simulink model "afe_dq_ttype"  (R2026b)
settings: Solver=ode23tb  StopTime=param.sim.simlength  FixedStep=param.sim.tc  MaxStep=param.glb_time.tc
values from neighbouring files (symbols this model uses):
  param = struct()    [init_model.m]
undefined symbols (not defined in the file or in its folder): magnitude
libraries: fl_lib x281, nesl_utility x136, igbt_simple_2th_lib x12, single_phase_transformer_lib x3, discrete_time_low_pass_filter x1, threephase_inductor_lib x1, dclink_for_three_levels x1, three_phase_three_level_ttype_inverter_ideal_switch_based_model x1, three_phase_three_levels_PWM_modulator x1, three_phase_bridge_three_level_ttype_igbt_simple_2th x1, three_phase_voltage_with_frt_emulator_mfcn x1
(part 8 of 8)

== system afe_dq_ttype/afe_dq_mod1/AFE_control/afe_control/grid_voltage_phase_lock_loops/FHT-PLL/pll_stageA/filter_and_transformation/FHTbeta ==
  u : Inport
  Bus Selector : BusSelector  OutputSignals=output_pu_hat,output_pu_hat_dot
  C Caller : CCaller  FunctionName=first_harmonic_tracker_process_simulink  PortSpecificationStruct="%)30     .    B \\   8    (     @         %    \"     D    !     0         %  0 \"0    $    _    07)G3F%M90  4&]R=$YA;64 4V-O<&4     26YD97@     5'EP90      4VEZ90      27-';&]B86P   X    P    !@    @    $          4    (     0    ,    !         !   P!O=70 #@   #     &    \"     0         !0    @    !     P    $         $  # &]U=  .    .     8    (    !          %    \"     $    &     0         0  ...(+4988 chars)"
  Constant : Constant  Value=param.glb_time.ts_afe
  Constant1 : Constant  Value=14
  Constant4 : Constant  Value=param.afe.ctrl.fht.omega_fht
  Constant5 : Constant  Value=param.afe.ctrl.fht.delta_fht
  Constant6 : Constant  Value=param.afe.ctrl.fht.Ld_fht(1)
  Constant7 : Constant  Value=param.afe.ctrl.fht.Ld_fht(2)
  Data Type Conversion{1..2,6..9} (6 alike) : DataTypeConversion  OutDataTypeStr=single  SaturateOnIntegerOverflow=off  RndMeth=Floor
  Data Type Conversion10 : DataTypeConversion  OutDataTypeStr=double  SaturateOnIntegerOverflow=off  RndMeth=Floor
  Data Type Conversion3 : DataTypeConversion  OutDataTypeStr=uint8  SaturateOnIntegerOverflow=off  RndMeth=Floor
  Data Type Conversion4 : DataTypeConversion  OutDataTypeStr=double  SaturateOnIntegerOverflow=off  RndMeth=Floor
  Data Type Conversion5 : DataTypeConversion  OutDataTypeStr=uint8  SaturateOnIntegerOverflow=off  RndMeth=Floor
  Gain : Gain  Gain=1/param.afe.ctrl.fht.omega_fht
  Step : Step  Time=0.0125  InitialValue=1  FinalValue=0
  ud_hat : Outport
  uq_hat : Outport  Port=2
  wires:
  Gain/1 -> uq_hat/1
  Bus Selector/2 -> Data Type Conversion10/1  "<output_pu_hat_dot>"
  Data Type Conversion10/1 -> Gain/1
  Data Type Conversion4/1 -> ud_hat/1
  Data Type Conversion3/1 -> C Caller/1
  Data Type Conversion1/1 -> C Caller/3
  Data Type Conversion2/1 -> C Caller/2
  C Caller/1 -> Bus Selector/1
  Bus Selector/1 -> Data Type Conversion4/1  "<output_pu_hat>"
  Step/1 -> Data Type Conversion3/1
  u/1 -> Data Type Conversion2/1
  Constant/1 -> Data Type Conversion1/1
  Constant1/1 -> Data Type Conversion5/1
  Constant4/1 -> Data Type Conversion6/1
  Constant6/1 -> Data Type Conversion8/1
  Constant7/1 -> Data Type Conversion9/1
  Constant5/1 -> Data Type Conversion7/1
  Data Type Conversion5/1 -> C Caller/8
  Data Type Conversion6/1 -> C Caller/4
  Data Type Conversion7/1 -> C Caller/5
  Data Type Conversion8/1 -> C Caller/6
  Data Type Conversion9/1 -> C Caller/7

== system afe_dq_ttype/afe_dq_mod1/AFE_control/afe_control/grid_voltage_phase_lock_loops/FHT-PLL_simulink/pll_stageA/filter_and_transformation/FHTalpha ==
  u : Inport
  Gain : Gain  Gain=param.afe.ctrl.fht.Ld_fht  Multiplication=Matrix(K*u)
  Gain1 : Gain  Gain=param.afe.ctrl.fht.Ad_fht  Multiplication=Matrix(K*u)
  Gain2 : Gain  Gain=param.afe.ctrl.fht.Cfht  Multiplication=Matrix(K*u)
  Gain3 : Gain  Gain=1/param.afe.ctrl.fht.omega_fht
  Selector : Selector  InputPortWidth=2  IndexOptions=Index vector (dialog)  Indices=1  OutputSizes=1  RuntimeRangeChecks=off
  Selector1 : Selector  InputPortWidth=2  IndexOptions=Index vector (dialog)  Indices=2  OutputSizes=1  RuntimeRangeChecks=off
  Sum : Sum  Inputs=-+|
  Sum1 : Sum  Inputs=|++
  Unit Delay : UnitDelay  SampleTime=-1
  ualpha : Outport
  ubeta : Outport  Port=2
  wires:
  u/1 -> Sum/2
  Unit Delay/1 -> Gain2/1, Selector1/1, Selector/1, Gain1/1
  Sum/1 -> Gain/1
  Sum1/1 -> Unit Delay/1
  Gain1/1 -> Sum1/2
  Gain2/1 -> Sum/1
  Selector/1 -> ualpha/1
  Gain/1 -> Sum1/1
  Selector1/1 -> Gain3/1
  Gain3/1 -> ubeta/1

== system afe_dq_ttype/afe_dq_mod1/AFE_control/afe_control/grid_voltage_phase_lock_loops/FHT-PLL_simulink/pll_stageA/filter_and_transformation/FHTbeta ==
  u : Inport
  Gain : Gain  Gain=param.afe.ctrl.fht.Ld_fht  Multiplication=Matrix(K*u)
  Gain1 : Gain  Gain=param.afe.ctrl.fht.Ad_fht  Multiplication=Matrix(K*u)
  Gain2 : Gain  Gain=param.afe.ctrl.fht.Cfht  Multiplication=Matrix(K*u)
  Gain3 : Gain  Gain=1/param.afe.ctrl.fht.omega_fht
  Selector : Selector  InputPortWidth=2  IndexOptions=Index vector (dialog)  Indices=1  OutputSizes=1  RuntimeRangeChecks=off
  Selector1 : Selector  InputPortWidth=2  IndexOptions=Index vector (dialog)  Indices=2  OutputSizes=1  RuntimeRangeChecks=off
  Sum : Sum  Inputs=-+|
  Sum1 : Sum  Inputs=|++
  Unit Delay : UnitDelay  SampleTime=-1
  ualpha : Outport
  ubeta : Outport  Port=2
  wires:
  Gain3/1 -> ubeta/1
  Selector1/1 -> Gain3/1
  Gain/1 -> Sum1/1
  Selector/1 -> ualpha/1
  Gain2/1 -> Sum/1
  Gain1/1 -> Sum1/2
  Sum1/1 -> Unit Delay/1
  Sum/1 -> Gain/1
  Unit Delay/1 -> Gain1/1, Selector/1, Selector1/1, Gain2/1
  u/1 -> Sum/2

== system afe_dq_ttype/afe_dq_mod1/AFE_control/afe_control/grid_voltage_phase_lock_loops/dq_pll/pll_stageA/sequences/alphabeta2xieta ==
  alpha : Inport
  beta : Inport  Port=2
  gamma : Inport  Port=3
  alphabeta2xieta_neg : MATLAB Function  TreatAsAtomicUnit=on
  alphabeta2xieta_pos : MATLAB Function  TreatAsAtomicUnit=on
  xi : Outport
  eta : Outport  Port=2
  Out3 : Outport  Port=3
  Out4 : Outport  Port=4
  wires:
  alpha/1 -> alphabeta2xieta_neg/1(alpha), alphabeta2xieta_pos/1(alpha)  "u_grid_alpha"
  beta/1 -> alphabeta2xieta_neg/2(beta), alphabeta2xieta_pos/2(beta)  "u_grid_beta"
  gamma/1 -> alphabeta2xieta_neg/3(gamma), alphabeta2xieta_pos/3(gamma)  "phase_grid"
  alphabeta2xieta_pos/1(xi) -> xi/1  "u_grid_pos_xi"
  alphabeta2xieta_pos/2(eta) -> eta/1  "u_grid_pos_eta"
  alphabeta2xieta_neg/1(xi) -> Out3/1  "u_grid_neg_xi"
  alphabeta2xieta_neg/2(eta) -> Out4/1  "u_grid_neg_eta"

== matlab function afe_dq_ttype/afe_dq_mod1/AFE_control/afe_control/grid_voltage_phase_lock_loops/FHT-PLL_simulink/pll_stageA/filter_and_transformation/abc2alphabeta ==
  data: a input; alpha output; b input; c input; beta output
function [alpha,beta] = abc2alphabeta(a,b,c)

alpha = 2/3*(a - 1/2*b - 1/2*c);
beta  = 1/sqrt(3)*(b - c);

end

== matlab function afe_dq_ttype/afe_dq_mod1/AFE_control/afe_control/grid_voltage_phase_lock_loops/FHT-PLL_simulink/pll_stageA/sequences/alphabeta2xieta ==
  data: alpha input; xi output; beta input; gamma input; eta output
function [xi,eta] = alphabeta2xieta_pos(alpha,beta,gamma)

    xi  =  (alpha*cos(gamma) + beta*sin(gamma));
    eta = (-alpha*sin(gamma) + beta*cos(gamma));

end

== matlab function afe_dq_ttype/afe_dq_mod1/AFE_control/afe_control/grid_voltage_phase_lock_loops/FHT-PLL_simulink/pll_stageB/bounder1 ==
  data: u input; y output
function y = bounder(u)
    y = -pi + mod(u+3*pi,2*pi);
end

== matlab function afe_dq_ttype/afe_dq_mod1/AFE_control/afe_control/grid_voltage_phase_lock_loops/FHT-PLL_simulink/pll_stageB/double_integrator_observer/bounder1 ==
  data: u input; y output
function y = bounder(u)
    
    y = -pi + mod(u+3*pi,2*pi);
    
end

== matlab function afe_dq_ttype/afe_dq_mod1/AFE_control/afe_control/grid_voltage_phase_lock_loops/dq_pll/pll_stageA/mormalization_and_transformation/abc2alphabeta ==
  data: a input; alpha output; b input; c input; beta output
function [alpha,beta] = abc2alphabeta(a,b,c)

alpha = 2/3*(a - 1/2*b - 1/2*c);
beta  = 1/sqrt(3)*(b - c);

end

== matlab function afe_dq_ttype/afe_dq_mod1/AFE_control/afe_control/grid_voltage_phase_lock_loops/dq_pll/pll_stageA/sequences/alphabeta2xieta/alphabeta2xieta_neg ==
  data: alpha input; xi output; beta input; gamma input; eta output
function [xi,eta] = alphabeta2xieta_neg(alpha,beta,gamma)

    xi  = alpha*cos(gamma) - beta*sin(gamma);
    eta = alpha*sin(gamma) + beta*cos(gamma);

end

== matlab function afe_dq_ttype/afe_dq_mod1/AFE_control/afe_control/grid_voltage_phase_lock_loops/dq_pll/pll_stageA/sequences/alphabeta2xieta/alphabeta2xieta_pos ==
  data: alpha input; xi output; beta input; gamma input; eta output
function [xi,eta] = alphabeta2xieta_pos(alpha,beta,gamma)

    xi  =  alpha*cos(gamma) + beta*sin(gamma);
    eta = -alpha*sin(gamma) + beta*cos(gamma);

end

== matlab function afe_dq_ttype/afe_dq_mod1/AFE_control/afe_control/grid_voltage_phase_lock_loops/dq_pll/pll_stageB/double_integrator_observer/bounder1 ==
  data: u input; y output
function y = bounder(u)
    
    y = -pi + mod(u+3*pi,2*pi);
    
end

== matlab function afe_dq_ttype/afe_dq_mod1/AFE_control/afe_control/grid_voltage_phase_lock_loops/dq_pll/pll_stageB/double_integrator_observer/bounder2 ==
  data: u input; y output
function y = bounder(u)
    
    y = -pi + mod(u+3*pi,2*pi);
    
end

== matlab function afe_dq_ttype/grid/power meter iec mfunc/three_phase_power_meter_iec ==
  data: phase input; m output Bus: PowerMeterIecBus; u_abc input; i_abc input; omega input; ts input; enable_time input
function m = three_phase_power_meter_iec(phase, u_abc, i_abc, omega, ts, enable_time)
%#codegen
% THREE_PHASE_POWER_METER_IEC
% Equivalente in singolo blocco MATLAB Function del sottosistema Simulink
% "three_phase_power_meter_iec" (libreria power_meter_iec).
%
% INGRESSI
%   phase       : angolo del PLL [rad]      (scalare)
%   u_abc       : tensioni di fase [V]      (3x1)
%   i_abc       : correnti di linea [A]     (3x1)
%   omega       : pulsazione di rete [rad/s] (scalare)
%   ts          : passo di campionamento [s]  -> parametro di maschera
%   enable_time : istante di abilitazione [s] -> parametro di maschera
%
% USCITA
%   m : struct (bus) con i campi, nello stesso ordine del Bus Creator
%       originale: Q1p, Q1n, P1n, P1p, U1n, U1p,
%                  i_act_1n, i_react_1n, i_act_1p, i_react_1p
%
% CATENA DI ELABORAZIONE (identica all'originale)
%   1) proiezione di ogni fase su cos(phase) e sin(phase), guadagno 2
%   2) media mobile dinamica su finestra pari a mezzo periodo di rete
%      (Tw = pi/|omega|), con lunghezza frazionaria interpolata
%   3) componenti simmetriche di sequenza diretta e inversa (Fortescue)
%   4) potenze attiva e reattiva per sequenza, tensioni concatenate RMS,
%      correnti attiva e reattiva per sequenza
%
% NOTE
%   - Il blocco deve girare a passo fisso ts (gli Zero-Order Hold di
%     ingresso dell'originale sono impliciti nel sample time del blocco).
%   - ts ed enable_time possono essere dichiarati come dati di scope
%     "Parameter" nel Symbols pane del MATLAB Function block, cosi'
%     risolvono direttamente sui parametri di maschera e la firma
%     esterna resta a 4 ingressi come nel blocco originale.

% ------------------------------------------------------------------
% Costanti
% ------------------------------------------------------------------
% MAVGFLT_SIZE_MAX = 17500;   % lunghezza buffer circolare (come originale)
MAVGFLT_SIZE_MAX = 2048;   % lunghezza buffer ridotto
NCH              = 12;      % canali filtrati: 6 per u_abc, 6 per i_abc

% Ordine canali:
%   1..3  ua_cos ub_cos uc_cos      7..9   ia_cos ib_cos ic_cos
%   4..6  ua_sin ub_sin uc_sin     10..12  ia_sin ib_sin ic_sin

% ------------------------------------------------------------------
% Stato persistente
% ------------------------------------------------------------------
persistent buf cb_index sample_count sum_short sum_long prev_input ...
           k_step period_held

if isempty(buf)
    buf          = zeros(NCH, MAVGFLT_SIZE_MAX);
    cb_index     = ones(NCH, 1);
    sample_count = ones(NCH, 1);
    sum_short    = zeros(NCH, 1);
    sum_long     = zeros(NCH, 1);
    prev_input   = zeros(NCH, 1);
    k_step       = 0;
    period_held  = 0;          % uscita iniziale dell'Enabled Subsystem
end

% ------------------------------------------------------------------
% Abilitazione (equivalente al blocco Step con Time = enable_time)
% ------------------------------------------------------------------
t_now  = k_step * ts;
k_step = k_step + 1;
enable = (t_now >= enable_time);

% ------------------------------------------------------------------
% Finestra di media: Enabled Subsystem 2*pi/w, alimentato da 2*|omega|.
% Quando |omega| = 0 l'Enabled Subsystem mantiene l'ultimo valore.
% ------------------------------------------------------------------
w2 = 2 * abs(omega);
if w2 > 0
    period_held = 2*pi / w2;   % = pi/|omega|, mezzo periodo di rete
end
period = period_held;

% ------------------------------------------------------------------
% Proiezione sin/cos, guadagno 2
% ------------------------------------------------------------------
c = cos(phase);
s = sin(phase);

x = zeros(NCH, 1);
x(1)  = 2 * u_abc(1) * c;   x(2)  = 2 * u_abc(2) * c;   x(3)  = 2 * u_abc(3) * c;
x(4)  = 2 * u_abc(1) * s;   x(5)  = 2 * u_abc(2) * s;   x(6)  = 2 * u_abc(3) * s;
x(7)  = 2 * i_abc(1) * c;   x(8)  = 2 * i_abc(2) * c;   x(9)  = 2 * i_abc(3) * c;
x(10) = 2 * i_abc(1) * s;   x(11) = 2 * i_abc(2) * s;   x(12) = 2 * i_abc(3) * s;

% ------------------------------------------------------------------
% Banco di 12 filtri a media mobile dinamica (dmavgflt_process)
% ------------------------------------------------------------------
y = zeros(NCH, 1);

if enable && period > 0

    desired = period / ts;
    if desired > (MAVGFLT_SIZE_MAX - 1)
        desired = MAVGFLT_SIZE_MAX - 1;
    end

    n_samples = floor(desired + 1);          % campioni che coprono il periodo
    frac      = desired + 1 - n_samples;     % parte frazionaria
    if n_samples < 1
        n_samples = 1;
    end

    for ch = 1:NCH

        ci = cb_index(ch);
        sc = sample_count(ch);

        if n_samples > sc
            % finestra in crescita: aggiungi campioni
            sum_short(ch) = sum_short(ch) + prev_input(ch);
            sum_long(ch)  = sum_long(ch)  + x(ch);
            sc = sc + 1;

        elseif n_samples < sc
            % finestra in contrazione: rimuovi i due campioni piu' vecchi
            i1 = mod(ci - 1 - sc,       MAVGFLT_SIZE_MAX) + 1;
            i2 = mod(ci - 1 - (sc - 1), MAVGFLT_SIZE_MAX) + 1;
            old_sum = buf(ch, i1) + buf(ch, i2);

            sum_short(ch) = sum_short(ch) + prev_input(ch) - old_sum;
            sum_long(ch)  = sum_long(ch)  + x(ch)          - old_sum;
            sc = sc - 1;

        else
            % finestra costante
            i1     = mod(ci - 1 - sc, MAVGFLT_SIZE_MAX) + 1;
            oldest = buf(ch, i1);

            sum_short(ch) = sum_short(ch) + prev_input(ch) - oldest;
            sum_long(ch)  = sum_long(ch)  + x(ch)          - oldest;
        end

        % aggiornamento buffer circolare
        buf(ch, ci)      = x(ch);
        cb_index(ch)     = mod(ci, MAVGFLT_SIZE_MAX) + 1;
        prev_input(ch)   = x(ch);
        sample_count(ch) = sc;

        % uscita: interpolazione lineare fra finestra corta e lunga
        if sc > 1
            avg_short = sum_short(ch) / (sc - 1);
        else
            avg_short = 0;
        end
        avg_long = sum_long(ch) / sc;

        y(ch) = avg_short * (1 - frac) + avg_long * frac;
    end
end
% se enable = false oppure period <= 0: y resta 0 e lo stato non evolve
% (comportamento identico all'originale)

ua_cos = y(1);  ub_cos = y(2);  uc_cos = y(3);
ua_sin = y(4);  ub_sin = y(5);  uc_sin = y(6);
ia_cos = y(7);  ib_cos = y(8);  ic_cos = y(9);
ia_sin = y(10); ib_sin = y(11); ic_sin = y(12);

% ------------------------------------------------------------------
% Componenti simmetriche (fasori con convenzione U = u_cos - j*u_sin)
% ------------------------------------------------------------------
sq3 = sqrt(3);

u1p_cos = (2*ua_cos - ub_cos - uc_cos - sq3*(uc_sin - ub_sin)) / 6;
u1p_sin = (2*ua_sin - ub_sin - uc_sin - sq3*(ub_cos - uc_cos)) / 6;
u1n_cos = (2*ua_cos - ub_cos - uc_cos - sq3*(ub_sin - uc_sin)) / 6;
u1n_sin = (2*ua_sin - ub_sin - uc_sin - sq3*(uc_cos - ub_cos)) / 6;

i1p_cos = (2*ia_cos - ib_cos - ic_cos - sq3*(ic_sin - ib_sin)) / 6;
i1p_sin = (2*ia_sin - ib_sin - ic_sin - sq3*(ib_cos - ic_cos)) / 6;
i1n_cos = (2*ia_cos - ib_cos - ic_cos - sq3*(ib_sin - ic_sin)) / 6;
i1n_sin = (2*ia_sin - ib_sin - ic_sin - sq3*(ic_cos - ib_cos)) / 6;

% ------------------------------------------------------------------
% Potenze per sequenza
% ------------------------------------------------------------------
P1p = 1.5 * (u1p_cos*i1p_cos + u1p_sin*i1p_sin);
Q1p = 1.5 * (u1p_cos*i1p_sin - u1p_sin*i1p_cos);
P1n = 1.5 * (u1n_cos*i1n_cos + u1n_sin*i1n_sin);
Q1n = 1.5 * (u1n_cos*i1n_sin - u1n_sin*i1n_cos);

% ------------------------------------------------------------------
% Tensioni concatenate RMS per sequenza: sqrt(3/2)*ampiezza di fase
% ------------------------------------------------------------------
U1p = sqrt(1.5 * (u1p_cos^2 + u1p_sin^2));
U1n = sqrt(1.5 * (u1n_cos^2 + u1n_sin^2));

% ------------------------------------------------------------------
% Correnti attiva e reattiva per sequenza (RMS di linea)
% La protezione contro la divisione per zero non era presente nello
% schema originale (i blocchi Divide restituivano Inf/NaN a U = 0).
% Portare U_MIN a 0 per replicare esattamente il comportamento vecchio.
% ------------------------------------------------------------------
U_MIN = 1e-9;

if U1p > U_MIN
    i_act_1p   = P1p / (sq3 * U1p);
    i_react_1p = Q1p / (sq3 * U1p);
else
    i_act_1p   = 0;
    i_react_1p = 0;
end

if U1n > U_MIN
    i_act_1n   = P1n / (sq3 * U1n);
    i_react_1n = Q1n / (sq3 * U1n);
else
    i_act_1n   = 0;
    i_react_1n = 0;
end

% ------------------------------------------------------------------
% Bus di uscita (stesso ordine dei campi dell'originale)
% ------------------------------------------------------------------
m.Q1p        = Q1p;
m.Q1n        = Q1n;
m.P1n        = P1n;
m.P1p        = P1p;
m.U1n        = U1n;
m.U1p        = U1p;
m.i_act_1n   = i_act_1n;
m.i_react_1n = i_react_1n;
m.i_act_1p   = i_act_1p;
m.i_react_1p = i_react_1p;

end

== matlab function afe_dq_ttype/afe_dq_mod1/AFE_control/afe_control/current_ctrl/xi_eta_to_alpha_beta ==
  data: xi input; alpha output; eta input; phase input; beta output
function [alpha,beta] = xi_eta_to_alpha_beta(xi,eta,phase)

    alpha = xi*cos(phase) - eta*sin(phase);
    beta  = xi*sin(phase) + eta*cos(phase);

end

== matlab function afe_dq_ttype/afe_dq_mod1/AFE_control/afe_control/grid_voltage_phase_lock_loops/dq_pll/pll_stageB/bounder1 ==
  data: u input; y output
function y = bounder(u)
    y = -pi + mod(u+3*pi,2*pi);
end

== matlab function afe_dq_ttype/afe_dq_mod1/AFE_control/afe_control/grid_voltage_phase_lock_loops/FHT-PLL_simulink/pll_stageB/double_integrator_observer/bounder2 ==
  data: u input; y output
function y = bounder(u)
    
    y = -pi + mod(u+3*pi,2*pi);
    
end

== matlab function afe_dq_ttype/afe_dq_mod1/afe/deadtime_generator_for_ttype/dead_time_generator_cmos_simulink_phu/dead_time_leg_generator_1/MATLAB Function ==
  data: u input; y output; Vpos_rail_dtg parameter
function y = not_cmos(u, Vpos_rail_dtg)

vth = Vpos_rail_dtg/2;

if u > vth
    y = 0;
else
    y = Vpos_rail_dtg;
end

== matlab function afe_dq_ttype/afe_dq_mod1/afe/deadtime_generator_for_ttype/dead_time_generator_cmos_simulink_phu/dead_time_leg_generator_1/MATLAB Function1 ==
  data: u1 input; u2 input; y output; Vpos_rail_dtg parameter
function y = and_cmos(u1, u2, Vpos_rail_dtg)

vth = Vpos_rail_dtg/2;

if (u1 > vth && u2 > vth)
    y = Vpos_rail_dtg;
else
    y = 0;
end

== matlab function afe_dq_ttype/afe_dq_mod1/afe/deadtime_generator_for_ttype/dead_time_generator_cmos_simulink_phu/dead_time_leg_generator_1/MATLAB Function2 ==
  data: u input; y output; Vpos_rail_dtg parameter
function y = not_cmos(u, Vpos_rail_dtg)

vth = Vpos_rail_dtg/2;

if u > vth
    y = 0;
else
    y = Vpos_rail_dtg;
end

== matlab function afe_dq_ttype/afe_dq_mod1/afe/deadtime_generator_for_ttype/dead_time_generator_cmos_simulink_phu/dead_time_leg_generator_1/MATLAB Function3 ==
  data: u input; y output; Vpos_rail_dtg parameter
function y = not_cmos(u, Vpos_rail_dtg)

vth = Vpos_rail_dtg/2;

if u > vth
    y = 0;
else
    y = Vpos_rail_dtg;
end

== matlab function afe_dq_ttype/afe_dq_mod1/afe/deadtime_generator_for_ttype/dead_time_generator_cmos_simulink_phu/dead_time_leg_generator_1/MATLAB Function4 ==
  data: u1 input; u2 input; y output; Vpos_rail_dtg parameter
function y = and_cmos(u1, u2, Vpos_rail_dtg)

vth = Vpos_rail_dtg/2;

if (u1 > vth && u2 > vth)
    y = Vpos_rail_dtg;
else
    y = 0;
end

== matlab function afe_dq_ttype/afe_dq_mod1/afe/deadtime_generator_for_ttype/dead_time_generator_cmos_simulink_phu/dead_time_leg_generator_1/MATLAB Function5 ==
  data: u1 input; u2 input; y output; Vpos_rail_dtg parameter
function y = and_cmos(u1, u2, Vpos_rail_dtg)

vth = Vpos_rail_dtg/2;

if (u1 > vth && u2 > vth)
    y = Vpos_rail_dtg;
else
    y = 0;
end

== matlab function afe_dq_ttype/afe_dq_mod1/afe/deadtime_generator_for_ttype/dead_time_generator_cmos_simulink_phu/dead_time_leg_generator_1/MATLAB Function6 ==
  data: u input; y output; Vpos_rail_dtg parameter
function y = not_cmos(u, Vpos_rail_dtg)

vth = Vpos_rail_dtg/2;

if u > vth
    y = 0;
else
    y = Vpos_rail_dtg;
end

== matlab function afe_dq_ttype/afe_dq_mod1/afe/deadtime_generator_for_ttype/dead_time_generator_cmos_simulink_phu/dead_time_leg_generator_1/MATLAB Function7 ==
  data: u input; y output; Vpos_rail_dtg parameter
function y = not_cmos(u, Vpos_rail_dtg)

vth = Vpos_rail_dtg/2;

if u > vth
    y = 0;
else
    y = Vpos_rail_dtg;
end

== matlab function afe_dq_ttype/afe_dq_mod1/afe/deadtime_generator_for_ttype/dead_time_generator_cmos_simulink_phu/dead_time_leg_generator_1/MATLAB Function8 ==
  data: u input; y output; Vpos_rail_dtg parameter
function y = not_cmos(u, Vpos_rail_dtg)

vth = Vpos_rail_dtg/2;

if u > vth
    y = 0;
else
    y = Vpos_rail_dtg;
end

== matlab function afe_dq_ttype/afe_dq_mod1/afe/deadtime_generator_for_ttype/dead_time_generator_cmos_simulink_phu/dead_time_leg_generator_1/MATLAB Function9 ==
  data: u1 input; u2 input; y output; Vpos_rail_dtg parameter
function y = and_cmos(u1, u2, Vpos_rail_dtg)

vth = Vpos_rail_dtg/2;

if (u1 > vth && u2 > vth)
    y = Vpos_rail_dtg;
else
    y = 0;
end

== matlab function afe_dq_ttype/afe_dq_mod1/afe/deadtime_generator_for_ttype/dead_time_generator_cmos_simulink_phv/dead_time_leg_generator_1/MATLAB Function ==
  data: u input; y output; Vpos_rail_dtg parameter
function y = not_cmos(u, Vpos_rail_dtg)

vth = Vpos_rail_dtg/2;

if u > vth
    y = 0;
else
    y = Vpos_rail_dtg;
end

== matlab function afe_dq_ttype/afe_dq_mod1/afe/deadtime_generator_for_ttype/dead_time_generator_cmos_simulink_phv/dead_time_leg_generator_1/MATLAB Function1 ==
  data: u1 input; u2 input; y output; Vpos_rail_dtg parameter
function y = and_cmos(u1, u2, Vpos_rail_dtg)

vth = Vpos_rail_dtg/2;

if (u1 > vth && u2 > vth)
    y = Vpos_rail_dtg;
else
    y = 0;
end

== matlab function afe_dq_ttype/afe_dq_mod1/afe/deadtime_generator_for_ttype/dead_time_generator_cmos_simulink_phv/dead_time_leg_generator_1/MATLAB Function2 ==
  data: u input; y output; Vpos_rail_dtg parameter
function y = not_cmos(u, Vpos_rail_dtg)

vth = Vpos_rail_dtg/2;

if u > vth
    y = 0;
else
    y = Vpos_rail_dtg;
end

== matlab function afe_dq_ttype/afe_dq_mod1/afe/deadtime_generator_for_ttype/dead_time_generator_cmos_simulink_phv/dead_time_leg_generator_1/MATLAB Function3 ==
  data: u input; y output; Vpos_rail_dtg parameter
function y = not_cmos(u, Vpos_rail_dtg)

vth = Vpos_rail_dtg/2;

if u > vth
    y = 0;
else
    y = Vpos_rail_dtg;
end

== matlab function afe_dq_ttype/afe_dq_mod1/afe/deadtime_generator_for_ttype/dead_time_generator_cmos_simulink_phv/dead_time_leg_generator_1/MATLAB Function4 ==
  data: u1 input; u2 input; y output; Vpos_rail_dtg parameter
function y = and_cmos(u1, u2, Vpos_rail_dtg)

vth = Vpos_rail_dtg/2;

if (u1 > vth && u2 > vth)
    y = Vpos_rail_dtg;
else
    y = 0;
end

== matlab function afe_dq_ttype/afe_dq_mod1/afe/deadtime_generator_for_ttype/dead_time_generator_cmos_simulink_phv/dead_time_leg_generator_1/MATLAB Function5 ==
  data: u1 input; u2 input; y output; Vpos_rail_dtg parameter
function y = and_cmos(u1, u2, Vpos_rail_dtg)

vth = Vpos_rail_dtg/2;

if (u1 > vth && u2 > vth)
    y = Vpos_rail_dtg;
else
    y = 0;
end

== matlab function afe_dq_ttype/afe_dq_mod1/afe/deadtime_generator_for_ttype/dead_time_generator_cmos_simulink_phv/dead_time_leg_generator_1/MATLAB Function6 ==
  data: u input; y output; Vpos_rail_dtg parameter
function y = not_cmos(u, Vpos_rail_dtg)

vth = Vpos_rail_dtg/2;

if u > vth
    y = 0;
else
    y = Vpos_rail_dtg;
end

== matlab function afe_dq_ttype/afe_dq_mod1/afe/deadtime_generator_for_ttype/dead_time_generator_cmos_simulink_phv/dead_time_leg_generator_1/MATLAB Function7 ==
  data: u input; y output; Vpos_rail_dtg parameter
function y = not_cmos(u, Vpos_rail_dtg)

vth = Vpos_rail_dtg/2;

if u > vth
    y = 0;
else
    y = Vpos_rail_dtg;
end

== matlab function afe_dq_ttype/afe_dq_mod1/afe/deadtime_generator_for_ttype/dead_time_generator_cmos_simulink_phv/dead_time_leg_generator_1/MATLAB Function8 ==
  data: u input; y output; Vpos_rail_dtg parameter
function y = not_cmos(u, Vpos_rail_dtg)

vth = Vpos_rail_dtg/2;

if u > vth
    y = 0;
else
    y = Vpos_rail_dtg;
end

== matlab function afe_dq_ttype/afe_dq_mod1/afe/deadtime_generator_for_ttype/dead_time_generator_cmos_simulink_phv/dead_time_leg_generator_1/MATLAB Function9 ==
  data: u1 input; u2 input; y output; Vpos_rail_dtg parameter
function y = and_cmos(u1, u2, Vpos_rail_dtg)

vth = Vpos_rail_dtg/2;

if (u1 > vth && u2 > vth)
    y = Vpos_rail_dtg;
else
    y = 0;
end

== matlab function afe_dq_ttype/afe_dq_mod1/afe/deadtime_generator_for_ttype/dead_time_generator_cmos_simulink_phw/dead_time_leg_generator_1/MATLAB Function ==
  data: u input; y output; Vpos_rail_dtg parameter
function y = not_cmos(u, Vpos_rail_dtg)

vth = Vpos_rail_dtg/2;

if u > vth
    y = 0;
else
    y = Vpos_rail_dtg;
end

== matlab function afe_dq_ttype/afe_dq_mod1/afe/deadtime_generator_for_ttype/dead_time_generator_cmos_simulink_phw/dead_time_leg_generator_1/MATLAB Function1 ==
  data: u1 input; u2 input; y output; Vpos_rail_dtg parameter
function y = and_cmos(u1, u2, Vpos_rail_dtg)

vth = Vpos_rail_dtg/2;

if (u1 > vth && u2 > vth)
    y = Vpos_rail_dtg;
else
    y = 0;
end

== matlab function afe_dq_ttype/afe_dq_mod1/afe/deadtime_generator_for_ttype/dead_time_generator_cmos_simulink_phw/dead_time_leg_generator_1/MATLAB Function2 ==
  data: u input; y output; Vpos_rail_dtg parameter
function y = not_cmos(u, Vpos_rail_dtg)

vth = Vpos_rail_dtg/2;

if u > vth
    y = 0;
else
    y = Vpos_rail_dtg;
end

== matlab function afe_dq_ttype/afe_dq_mod1/afe/deadtime_generator_for_ttype/dead_time_generator_cmos_simulink_phw/dead_time_leg_generator_1/MATLAB Function3 ==
  data: u input; y output; Vpos_rail_dtg parameter
function y = not_cmos(u, Vpos_rail_dtg)

vth = Vpos_rail_dtg/2;

if u > vth
    y = 0;
else
    y = Vpos_rail_dtg;
end

== matlab function afe_dq_ttype/afe_dq_mod1/afe/deadtime_generator_for_ttype/dead_time_generator_cmos_simulink_phw/dead_time_leg_generator_1/MATLAB Function4 ==
  data: u1 input; u2 input; y output; Vpos_rail_dtg parameter
function y = and_cmos(u1, u2, Vpos_rail_dtg)

vth = Vpos_rail_dtg/2;

if (u1 > vth && u2 > vth)
    y = Vpos_rail_dtg;
else
    y = 0;
end

== matlab function afe_dq_ttype/afe_dq_mod1/afe/deadtime_generator_for_ttype/dead_time_generator_cmos_simulink_phw/dead_time_leg_generator_1/MATLAB Function5 ==
  data: u1 input; u2 input; y output; Vpos_rail_dtg parameter
function y = and_cmos(u1, u2, Vpos_rail_dtg)

vth = Vpos_rail_dtg/2;

if (u1 > vth && u2 > vth)
    y = Vpos_rail_dtg;
else
    y = 0;
end

== matlab function afe_dq_ttype/afe_dq_mod1/afe/deadtime_generator_for_ttype/dead_time_generator_cmos_simulink_phw/dead_time_leg_generator_1/MATLAB Function6 ==
  data: u input; y output; Vpos_rail_dtg parameter
function y = not_cmos(u, Vpos_rail_dtg)

vth = Vpos_rail_dtg/2;

if u > vth
    y = 0;
else
    y = Vpos_rail_dtg;
end

== matlab function afe_dq_ttype/afe_dq_mod1/afe/deadtime_generator_for_ttype/dead_time_generator_cmos_simulink_phw/dead_time_leg_generator_1/MATLAB Function7 ==
  data: u input; y output; Vpos_rail_dtg parameter
function y = not_cmos(u, Vpos_rail_dtg)

vth = Vpos_rail_dtg/2;

if u > vth
    y = 0;
else
    y = Vpos_rail_dtg;
end

== matlab function afe_dq_ttype/afe_dq_mod1/AFE_control/afe_control/grid_voltage_phase_lock_loops/FHT-PLL/pll_stageA/filter_and_transformation/abc2alphabeta ==
  data: a input; alpha output; b input; c input; beta output
function [alpha,beta] = abc2alphabeta(a,b,c)

alpha = 2/3*(a - 1/2*b - 1/2*c);
beta  = 1/sqrt(3)*(b - c);

end

== matlab function afe_dq_ttype/afe_dq_mod1/afe/deadtime_generator_for_ttype/dead_time_generator_cmos_simulink_phw/dead_time_leg_generator_1/MATLAB Function8 ==
  data: u input; y output; Vpos_rail_dtg parameter
function y = not_cmos(u, Vpos_rail_dtg)

vth = Vpos_rail_dtg/2;

if u > vth
    y = 0;
else
    y = Vpos_rail_dtg;
end

== matlab function afe_dq_ttype/afe_dq_mod1/afe/deadtime_generator_for_ttype/dead_time_generator_cmos_simulink_phw/dead_time_leg_generator_1/MATLAB Function9 ==
  data: u1 input; u2 input; y output; Vpos_rail_dtg parameter
function y = and_cmos(u1, u2, Vpos_rail_dtg)

vth = Vpos_rail_dtg/2;

if (u1 > vth && u2 > vth)
    y = Vpos_rail_dtg;
else
    y = 0;
end

== matlab function afe_dq_ttype/afe_dq_mod1/AFE_control/afe_control/grid_voltage_phase_lock_loops/FHT-PLL/pll_stageA/sequences/alphabeta2xieta ==
  data: alpha input; xi output; beta input; gamma input; eta output
function [xi,eta] = alphabeta2xieta_pos(alpha,beta,gamma)

    xi  =  (alpha*cos(gamma) + beta*sin(gamma));
    eta = (-alpha*sin(gamma) + beta*cos(gamma));

end

== matlab function afe_dq_ttype/afe_dq_mod1/AFE_control/afe_control/current_ctrl/current_transformation/uvw2alphabeta ==
  data: u input; alpha output; v input; w input; beta output
function [alpha,beta] = uvw2alphabeta(u,v,w)

alpha = 2/3*(u - 1/2*v - 1/2*w);
beta  = 2/3*(sqrt(3)/2*(v - w));

end

== matlab function afe_dq_ttype/afe_dq_mod1/AFE_control/afe_control/current_ctrl/current_transformation/alphabeta2xieta ==
  data: alpha input; xi output; beta input; gamma input; eta output
function [xi,eta] = alphabeta2xieta(alpha,beta,gamma)

    xi  =  alpha*cos(gamma) + beta*sin(gamma);
    eta = -alpha*sin(gamma) + beta*cos(gamma);

end

== matlab function afe_dq_ttype/afe_dq_mod1/AFE_control/afe_control/grid_voltage_phase_lock_loops/FHT-PLL/pll_stageB/bounder1 ==
  data: u input; y output
function y = bounder(u)
    y = -pi + mod(u+3*pi,2*pi);
end

== matlab function afe_dq_ttype/afe_dq_mod1/AFE_control/afe_control/grid_voltage_phase_lock_loops/FHT-PLL/pll_stageB/double_integrator_observer/bounder1 ==
  data: u input; y output
function y = bounder(u)
    
    y = -pi + mod(u+3*pi,2*pi);
    
end

== matlab function afe_dq_ttype/afe_dq_mod1/AFE_control/afe_control/grid_voltage_phase_lock_loops/FHT-PLL/pll_stageB/double_integrator_observer/bounder2 ==
  data: u input; y output
function y = bounder(u)
    
    y = -pi + mod(u+3*pi,2*pi);
    
end
